simulink model "tank_control"  (R2026b)
settings: Solver=ode45  StopTime=p.t_end  MaxStep=0.1  RelTol=1e-6  AbsTol=1e-8
model workspace (MAT data in the model file):
  p.A = 0.05
  p.k_out = 0.0015
  p.h0 = 0.4
  p.r0 = 0.4
  p.r1 = 0.6
  p.t_ref = 20
  p.t_dist = 180
  p.dist_amp = 0.0003
  p.q_max = 0.004
  p.Kp = 0.004
  p.Ki = 0.00015
  p.Kd = 0.004
  p.N = 5
  p.Kaw = 0.2
  p.integral_enabled = 1
  p.t_end = 360
  p.q_bias = 0.000948683298051
settings Model: Creator=Rudraksha  LastModifiedBy=Rudraksha
settings DataIOCC: SaveOutput=off  SaveTime=off  SignalLogging=off

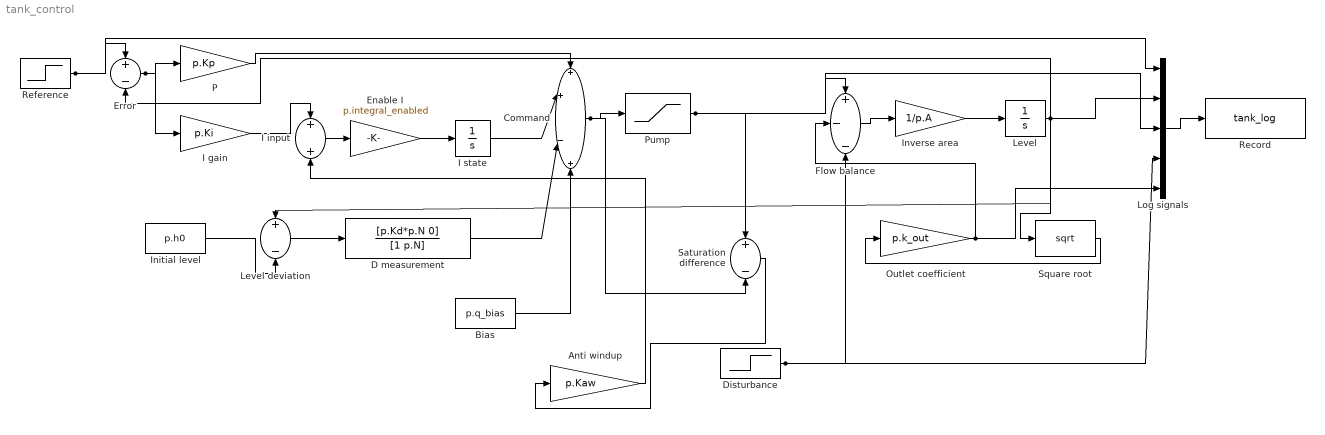
== system tank_control ==
  Anti windup : Gain  Gain=p.Kaw
  Bias : Constant  Value=p.q_bias
  Command : Sum  Inputs=++-+
  D measurement : TransferFcn  Numerator=[p.Kd*p.N 0]  Denominator=[1 p.N]
  Disturbance : Step  Time=p.t_dist  FinalValue=p.dist_amp  SampleTime=0
  Enable I : Gain  Gain=p.integral_enabled
  Error : Sum  Inputs=+-
  Flow balance : Sum  Inputs=+--
  I gain : Gain  Gain=p.Ki
  I input : Sum
  I state : Integrator
  Initial level : Constant  Value=p.h0
  Inverse area : Gain  Gain=1/p.A
  Level : Integrator  InitialCondition=p.h0  LimitOutput=on  LowerSaturationLimit=0
  Level deviation : Sum  Inputs=+-
  Log signals : Mux  Inputs=5
  Outlet coefficient : Gain  Gain=p.k_out
  P : Gain  Gain=p.Kp
  Pump : Saturate  UpperLimit=p.q_max  LowerLimit=0
  Record : ToWorkspace  VariableName=tank_log  SaveFormat=Timeseries  SampleTime=-1
  Reference : Step  Time=p.t_ref  InitialValue=p.r0  FinalValue=p.r1  SampleTime=0
  Saturation difference : Sum  Inputs=+-
  Square root : Sqrt
  wires:
  Reference/1 -> Error/1, Log signals/1
  Level/1 -> Error/2, Level deviation/1, Square root/1, Log signals/2
  Error/1 -> P/1, I gain/1
  I gain/1 -> I input/1
  Anti windup/1 -> I input/2
  I input/1 -> Enable I/1
  Enable I/1 -> I state/1
  P/1 -> Command/1
  I state/1 -> Command/2
  Initial level/1 -> Level deviation/2
  Level deviation/1 -> D measurement/1
  D measurement/1 -> Command/3
  Bias/1 -> Command/4
  Command/1 -> Pump/1, Saturation difference/2
  Pump/1 -> Saturation difference/1, Flow balance/1, Log signals/3
  Saturation difference/1 -> Anti windup/1
  Outlet coefficient/1 -> Flow balance/2, Log signals/5
  Disturbance/1 -> Flow balance/3, Log signals/4
  Flow balance/1 -> Inverse area/1
  Inverse area/1 -> Level/1
  Square root/1 -> Outlet coefficient/1
  Log signals/1 -> Record/1
